simulink model "nonLinearPlant"  (R2026a)
settings: Solver=ode45

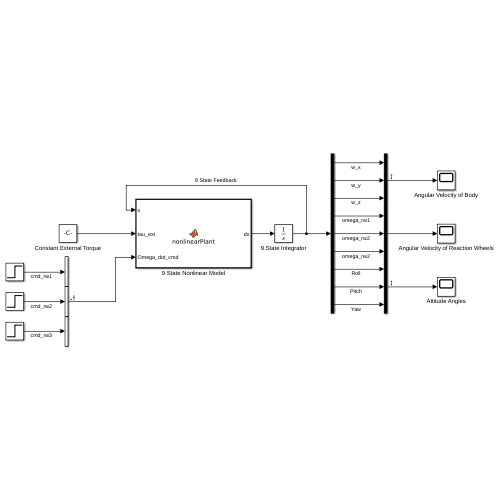
[thumbnail: Simulink's stored preview of the top-level diagram]
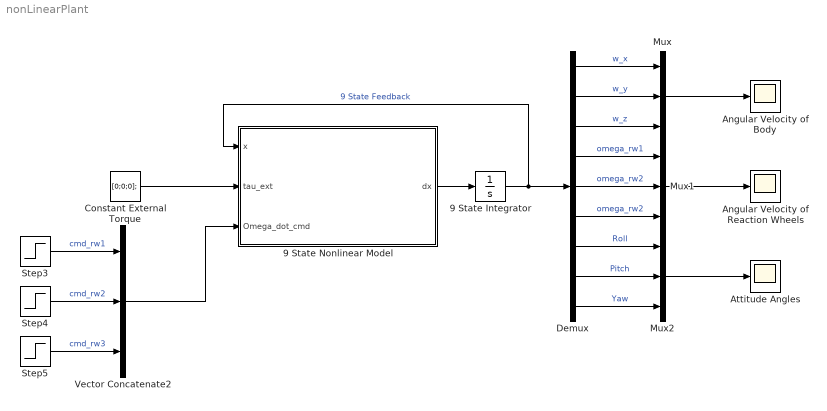
== system nonLinearPlant ==
  9 State Integrator : Integrator  InitialCondition=zeros(9,1)
  9 State Nonlinear Model : MATLAB Function  TreatAsAtomicUnit=on
  Angular Velocity of Body : Scope
      settings: ActiveDisplayYMinimum=-6.5088834764831862  ActiveDisplayYMaximum=8.5799512883486617
  Angular Velocity of Reaction Wheels : Scope
      settings: ActiveDisplayYMinimum=-1.2499999999999998  ActiveDisplayYMaximum=11.25
  Attitude Angles : Scope
      settings: ActiveDisplayYMinimum=-8.021240189198366  ActiveDisplayYMaximum=56.53405777075259  DataLoggingVariableName=ScopeData2
  Constant External Torque : Constant  Value=[0;0;0];
  Demux : Demux  Outputs=9
  Mux : Mux  Inputs=3
  Mux1 : Mux  Inputs=3
  Mux2 : Mux  Inputs=3
  Step3 : Step  FinalValue=0  SampleTime=0
  Step4 : Step  FinalValue=0  SampleTime=0
  Step5 : Step  FinalValue=0  SampleTime=0
  Vector Concatenate2 : Concatenate  NumInputs=3
  wires:
  Vector Concatenate2/1 -> 9 State Nonlinear Model/3(Omega_dot_cmd)
  Constant External Torque/1 -> 9 State Nonlinear Model/2(tau_ext)
  Step4/1 -> Vector Concatenate2/2  "cmd_rw2"
  Step5/1 -> Vector Concatenate2/3  "cmd_rw3"
  9 State Integrator/1 -> Demux/1, 9 State Nonlinear Model/1(x)  "9 State Feedback"
  9 State Nonlinear Model/1(dx) -> 9 State Integrator/1
  Demux/1 -> Mux/1  "w_x"
  Demux/2 -> Mux/2  "w_y"
  Demux/3 -> Mux/3  "w_z"
  Demux/4 -> Mux1/1  "omega_rw1"
  Demux/5 -> Mux1/2  "omega_rw2"
  Demux/6 -> Mux1/3  "omega_rw2"
  Mux/1 -> Angular Velocity of Body/1
  Mux1/1 -> Angular Velocity of Reaction Wheels/1
  Demux/7 -> Mux2/1  "Roll"
  Demux/8 -> Mux2/2  "Pitch"
  Demux/9 -> Mux2/3  "Yaw"
  Mux2/1 -> Attitude Angles/1
  Step3/1 -> Vector Concatenate2/1  "cmd_rw1"

== matlab function nonLinearPlant/9 State Nonlinear Model ==
  data: x input; dx output; tau_ext input; Omega_dot_cmd input
function dx = nonlinearPlant(x,tau_ext,Omega_dot_cmd)

    I = [1 0 0;
         0 1 0;
         0 0 1];
    
    I_rw = [1 0 0; 
            0 1 0;
            0 0 1];
    
    R_rw_b = [-sqrt(2)/2   1/2          1/2;
               0          -sqrt(2)/2    sqrt(2)/2;
               sqrt(2)/2   1/2          1/2];
    
    R_b_rw = transpose(R_rw_b);
    
    wx = x(1);
    wy = x(2);
    wz = x(3);
    
    Omega_x = x(4);
    Omega_y = x(5);
    Omega_z = x(6);
    
    phi   = x(7);
    theta = x(8);
    psi   = x(9);
    
    w = [wx;wy;wz];
    
    Omega = [Omega_x;Omega_y;Omega_z];
    
    Omega_dot = Omega_dot_cmd;
    
    w_dot = I \ ( ...
        tau_ext ...
        - cross(w,I*w) ...
        - R_b_rw*(I_rw*Omega_dot) ...
        - cross(w,R_b_rw*(I_rw*Omega)) );

   
    phi_dot = ...
        wx ...
        + wy*sin(phi)*tan(theta) ...
        + wz*cos(phi)*tan(theta);
    
    theta_dot = ...
        wy*cos(phi) ...
        - wz*sin(phi);
    
    psi_dot = ...
        (wy*sin(phi) ...
        + wz*cos(phi)) / cos(theta);
    
    dx = [
        w_dot;
        Omega_dot;
        phi_dot;
        theta_dot;
        psi_dot
    ];

end
